simulink model "EV_Charger_SinglePhase_G2V"  (R2024b)
settings: Solver=ode23t  StartTime=0.0  StopTime=1  FixedStep=1e-6  RelTol=1e-3
undefined symbols (not defined in the file): Ion, Lithium
libraries: spsSeriesRLCBranchLib x8, spsMosfetLib x6, spsCurrentMeasurementLib x3, spsVoltageMeasurementLib x3, slpidlib x3, spsPLLLib x1, spsACVoltageSourceLib x1, spsPWMGeneratorDCDCLib x1, spsPWMGenerator2LevelLib x1, spsBatteryLib x1, sps_lib x1
settings Model: Creator=SUDHAK1  LastModifiedBy=SUDHAK1

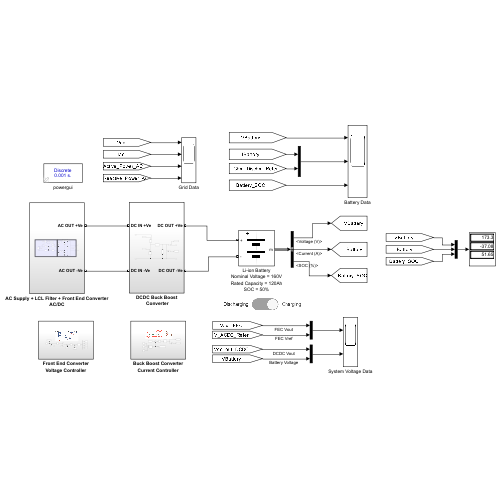
[thumbnail: Simulink's stored preview of the top-level diagram]
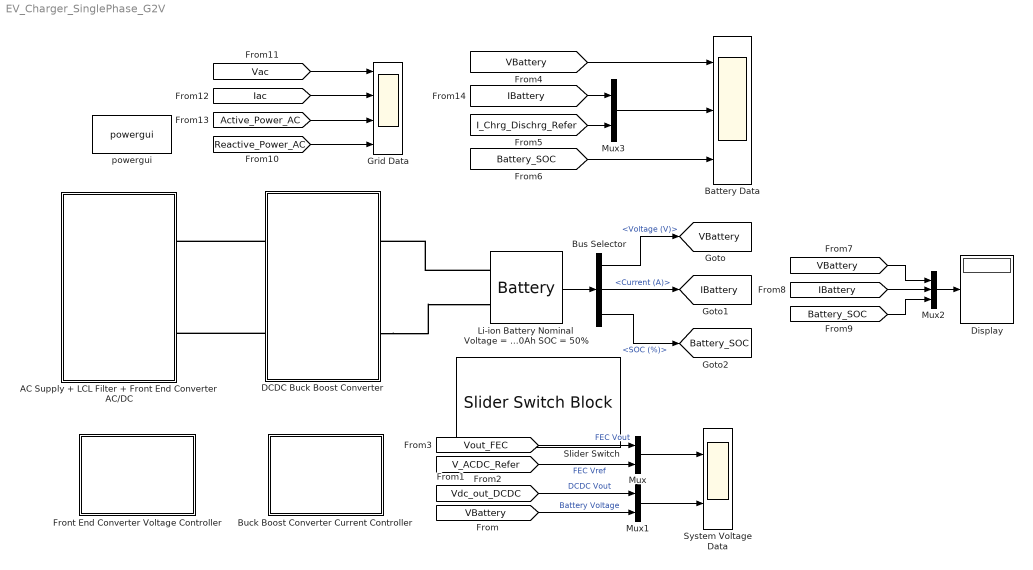
== system EV_Charger_SinglePhase_G2V ==
  AC Supply + LCL Filter + Front End Converter AC/DC : Subsystem
  Battery Data : Scope  NumInputPorts=3
  Buck Boost Converter Current Controller : Subsystem
  Bus Selector : BusSelector  OutputSignals=Voltage (V),Current (A),SOC (%)
  DCDC Buck Boost Converter : Subsystem
  Display : Display
  Front End Converter Voltage Controller : Subsystem
  Grid Data : Scope  NumInputPorts=4
  Li-ion Battery Nominal Voltage = 160V Rated Capacity = 120Ah SOC = 50% : spsBatteryLib/Battery  BatType=Lithium-Ion  NomV=160  NomQ=120  SOC=50  Batt_Tr=1  PresetModel=on  MaxQ=120  MinV=120  FullV=186.2379  Dis_rate=52.1739  R=0.013333  Normal_OP=108.5217  expZone="[172.8617      5.895652]"
  Mux : Mux  Inputs=2
  Mux1 : Mux  Inputs=2
  Mux2 : Mux  Inputs=3
  Mux3 : Mux  Inputs=2
  Slider Switch : SliderSwitchBlock  LabelPosition=Hide
      settings: Values={{'Discharging', 'Charging'}, [0 1]}
  System Voltage Data : Scope  NumInputPorts=2
  powergui : sps_lib/powergui  Priority=1  SimulationMode=Discrete  SampleTime=1e-3  frequency=60  Iterations=50  frequencyindice=50  Pbase=100e6  ErrMax=1e-4  UnitsV=kV  UnitsW=MW  buscounter=0  FunctionMessages=off  echomessages=off  EnableUseOfTLC=off  CurrentSourceSwitches=off  DisableSnubberDevices=off  DisableRonSwitches=off  DisableVfSwitches=off  DisplayEquations=off  AutomaticDiscreteSolvers=off  SolverType=Tustin/Backward Euler (TBE)  Interpol=off  ExternalGateDelay=off  methode=off  Ts=100  x0status=blocks  SPID=on  SwTol=0  HookPort=off  NonlinearTolerance=1e-4  nMaxIteration=100  ContinueOnMaxIteration=off  RestoreLinks=warning  ResistiveCurrentMeasurement=off  Frange=[0:2:500]  Ylog=off  Xlog=on  ShowGrid=off  save=off  variable=ZData  structure=0  ZoomFFT=off  StartTime=0.0  cycles=1  DisplayStyle=1  fundamental=60  FreqAxis=off  MaxFrequency=1000  frequencyindicesteady=1  RmsSteady=1  display=off
  tag scope: Battery_SOC=global, IBattery=global, VBattery=global
  wires:
  Li-ion Battery Nominal Voltage = 160V Rated Capacity = 120Ah SOC = 50%/1 -> Bus Selector/1
  Bus Selector/1 -> [VBattery]  "<Voltage (V)>"
  Bus Selector/2 -> [IBattery]  "<Current (A)>"
  Bus Selector/3 -> [Battery_SOC]  "<SOC (%)>"
  [VBattery] -> Mux2/1
  [Battery_SOC] -> Mux2/3
  [IBattery] -> Mux2/2
  Mux2/1 -> Display/1
  Mux/1 -> System Voltage Data/1
  [Vdc_out_DCDC] -> Mux1/1  "DCDC Vout"
  [VBattery] -> Mux1/2  "Battery Voltage"
  [V_ACDC_Refer] -> Mux/2  "FEC Vref"
  [Vout_FEC] -> Mux/1  "FEC Vout"
  [Reactive_Power_AC] -> Grid Data/4
  [VBattery] -> Battery Data/1
  [Vac] -> Grid Data/1
  [Battery_SOC] -> Battery Data/3
  [Active_Power_AC] -> Grid Data/3
  Mux1/1 -> System Voltage Data/2
  [Iac] -> Grid Data/2
  [IBattery] -> Mux3/1
  [I_Chrg_Dischrg_Refer] -> Mux3/2
  Mux3/1 -> Battery Data/2
  connections:
  Li-ion Battery Nominal Voltage = 160V Rated Capacity = 120Ah SOC = 50%/LConn1 -- DCDC Buck Boost Converter/RConn1
  DCDC Buck Boost Converter/RConn2 -- Li-ion Battery Nominal Voltage = 160V Rated Capacity = 120Ah SOC = 50%/LConn2
  DCDC Buck Boost Converter/LConn1 -- AC Supply + LCL Filter + Front End Converter AC/DC/RConn1
  DCDC Buck Boost Converter/LConn2 -- AC Supply + LCL Filter + Front End Converter AC/DC/RConn2

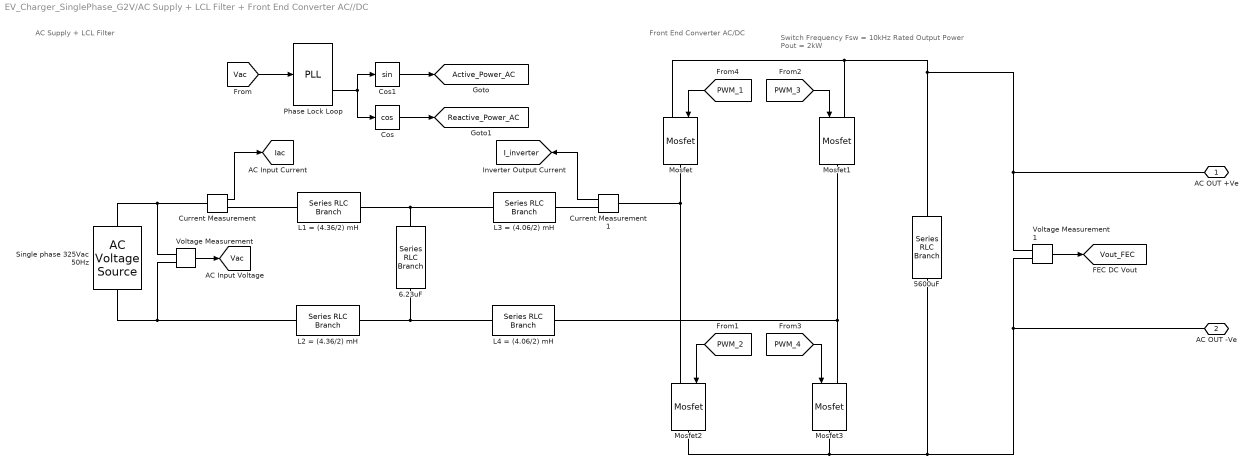
== system EV_Charger_SinglePhase_G2V/AC Supply + LCL Filter + Front End Converter AC//DC ==
  note: Front End Converter
      | AC/DC
  note: AC Supply + LCL Filter
  note: Switch Frequency Fsw = 10kHz
      | Rated Output Power Pout = 2kW
  5600uF : spsSeriesRLCBranchLib/Series RLC Branch  LConnTagsString=__new0  RConnTagsString=__new0  BranchType=RC  Resistance=0.0001  Inductance=1e-3  SetiL0=off  InitialCurrent=0  Capacitance=5600e-6  Setx0=on  InitialVoltage=400  Measurements=None
  6.23uF : spsSeriesRLCBranchLib/Series RLC Branch  LConnTagsString=__new0  RConnTagsString=__new0  BranchType=C  Resistance=1  Inductance=1e-3  SetiL0=off  InitialCurrent=0  Capacitance=6.23e-6  Setx0=off  InitialVoltage=0  Measurements=None
  Cos : Trigonometry  Operator=cos
  Cos1 : Trigonometry
  Current Measurement : spsCurrentMeasurementLib/Current Measurement  PhasorSimulation=off  OutputType=Complex  PSBequivalent=0
  Current Measurement1 : spsCurrentMeasurementLib/Current Measurement  PhasorSimulation=off  OutputType=Complex  PSBequivalent=0
  L1 = (4.36/2) mH : spsSeriesRLCBranchLib/Series RLC Branch  LConnTagsString=__new0  RConnTagsString=__new0  BranchType=L  Resistance=1  Inductance=4.36e-3/2  SetiL0=off  InitialCurrent=0  Capacitance=1e-6  Setx0=off  InitialVoltage=0  Measurements=None
  L2 = (4.36/2) mH : spsSeriesRLCBranchLib/Series RLC Branch  LConnTagsString=__new0  RConnTagsString=__new0  BranchType=L  Resistance=1  Inductance=4.36e-3/2  SetiL0=off  InitialCurrent=0  Capacitance=1e-6  Setx0=off  InitialVoltage=0  Measurements=None
  L3 = (4.06/2) mH : spsSeriesRLCBranchLib/Series RLC Branch  LConnTagsString=__new0  RConnTagsString=__new0  BranchType=L  Resistance=1  Inductance=4.06e-3/2  SetiL0=off  InitialCurrent=0  Capacitance=1e-6  Setx0=off  InitialVoltage=0  Measurements=None
  L4 = (4.06/2) mH : spsSeriesRLCBranchLib/Series RLC Branch  LConnTagsString=__new0  RConnTagsString=__new0  BranchType=L  Resistance=1  Inductance=4.06e-3/2  SetiL0=off  InitialCurrent=0  Capacitance=1e-6  Setx0=off  InitialVoltage=0  Measurements=None
  Mosfet{,1..3} (4 alike) : spsMosfetLib/Mosfet  Ron=0.1  Lon=0  Rd=0.01  Vfd=0  IC=0  Rs=1e5  Cs=inf  Measurements=off
  Phase Lock Loop : spsPLLLib/PLL  Fmin=45  Par_Init=[0, 50]  ParK=[180, 3200, 1]  TcD=1e-6  MaxRateChangeFreq=12  FilterCutOffFreq=25  Ts=0  AGC=on
      settings: LibrarySourceBlock=sps_lib/Control/PLL
  Single phase 325Vac 50Hz : spsACVoltageSourceLib/AC Voltage Source  Amplitude=325  Phase=0  Frequency=50  SampleTime=0  Measurements=None  BusType=swing  Pref=10e3  Qref=0  Qmin=-inf  Qmax=+inf
  Voltage Measurement : spsVoltageMeasurementLib/Voltage Measurement  PhasorSimulation=off  OutputType=Complex  PSBequivalent=0
  Voltage Measurement1 : spsVoltageMeasurementLib/Voltage Measurement  PhasorSimulation=off  OutputType=Complex  PSBequivalent=0
  AC OUT +Ve : PMIOPort  Side=Right
  AC OUT -Ve : PMIOPort  Port=2  Side=Right
  tag scope: Active_Power_AC=global, I_inverter=global, Iac=global, Reactive_Power_AC=global, Vac=global, Vout_FEC=global
  wires:
  Current Measurement1/1 -> [I_inverter]
  Current Measurement/1 -> [Iac]
  Voltage Measurement/1 -> [Vac]
  Voltage Measurement1/1 -> [Vout_FEC]
  [PWM_2] -> Mosfet2/1
  [PWM_1] -> Mosfet/1
  [PWM_3] -> Mosfet1/1
  [PWM_4] -> Mosfet3/1
  Phase Lock Loop/2 -> Cos1/1, Cos/1
  [Vac] -> Phase Lock Loop/1
  Cos/1 -> [Reactive_Power_AC]
  Cos1/1 -> [Active_Power_AC]
  connections:
  Current Measurement1/RConn1 -- L3 = (4.06/2) mH/RConn1
  Current Measurement/RConn1 -- L1 = (4.36/2) mH/LConn1
  L2 = (4.36/2) mH/RConn1 -- 6.23uF/RConn1 -- L4 = (4.06/2) mH/LConn1
  Single phase 325Vac 50Hz/LConn1 -- Voltage Measurement/LConn2 -- L2 = (4.36/2) mH/LConn1
  L1 = (4.36/2) mH/RConn1 -- 6.23uF/LConn1 -- L3 = (4.06/2) mH/LConn1
  Single phase 325Vac 50Hz/RConn1 -- Voltage Measurement/LConn1 -- Current Measurement/LConn1
  L4 = (4.06/2) mH/RConn1 -- Mosfet1/RConn1 -- Mosfet3/LConn1
  Current Measurement1/LConn1 -- Mosfet2/LConn1 -- Mosfet/RConn1
  5600uF/LConn1 -- Mosfet/LConn1 -- Mosfet1/LConn1 -- AC OUT +Ve/RConn1 -- Voltage Measurement1/LConn1
  5600uF/RConn1 -- Voltage Measurement1/LConn2 -- AC OUT -Ve/RConn1 -- Mosfet2/RConn1 -- Mosfet3/RConn1

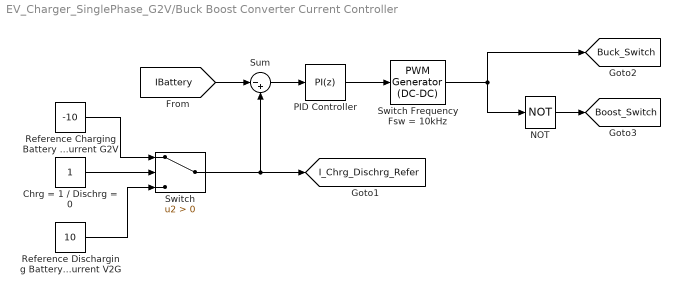
== system EV_Charger_SinglePhase_G2V/Buck Boost Converter Current Controller ==
  Chrg = 1 / Dischrg = 0 : Constant
  NOT : Logic  Operator=NOT  IconShape=distinctive  AllPortsSameDT=off  OutDataTypeStr=boolean
  PID Controller : slpidlib/PID Controller  Controller=PI  Form=Parallel  TimeDomain=Discrete-time  UseExternalTs=off  SampleTime=-1  IntegratorMethod=Forward Euler  FilterMethod=Forward Euler  ControllerParametersSource=internal  P=0.005  I=10  UseKiTs=off  D=0  UseExternalDerivativeSource=off  N=100  UseFilter=on  TunerSelectOption=Transfer Function Based (PID Tuner App)  InitialConditionSource=internal  InitialConditionForIntegrator=0  InitialConditionForFilter=0  DifferentiatorICPrevScaledInput=0  ExternalReset=none  TrackingMode=off  Kt=1  LimitOutput=on  SatLimitsSource=internal  UpperSaturationLimit=0.95  LowerSaturationLimit=0  LinearizeAsGain=on  AntiWindupMode=none  Kb=1  LimitIntegrator=off  UpperIntegratorSaturationLimit=inf  LowerIntegratorSaturationLimit=-inf  POutMin=[]  POutMax=[]  IOutMin=[]  IOutMax=[]  DOutMin=[]  DOutMax=[]  NOutMin=[]  NOutMax=[]  SumOutMin=[]  SumOutMax=[]  SaturationOutMin=[]  SaturationOutMax=[]  PParamMin=[]  PParamMax=[]  IParamMin=[]  IParamMax=[]  DParamMin=[]  DParamMax=[]  NParamMin=[]  NParamMax=[]  KbParamMin=[]  KbParamMax=[]  KtParamMin=[]  KtParamMax=[]  KbOutMin=[]  KbOutMax=[]  KtOutMin=[]  KtOutMax=[]  IntegratorOutMin=[]  IntegratorOutMax=[]  FilterOutMin=[]  FilterOutMax=[]  SumI1OutMin=[]  SumI1OutMax=[]  SumI2OutMin=[]  SumI2OutMax=[]  SumI3OutMin=[]  SumI3OutMax=[]  SumI4OutMin=[]  SumI4OutMax=[]  SumDOutMin=[]  SumDOutMax=[]  DifferentiatorOutMin=[]  DifferentiatorOutMax=[]  FilterDiffOutCoefMin=[]  FilterDiffOutCoefMax=[]  ReciprocalOutMin=[]  ReciprocalOutMax=[]  SumDenOutMin=[]  SumDenOutMax=[]  SumNumOutMin=[]  SumNumOutMax=[]  DivideOutMin=[]  DivideOutMax=[]  UdiffTsProdOutMin=[]  UdiffTsProdOutMax=[]  NTsProdOutMin=[]  NTsProdOutMax=[]  UintegralTsProdOutMin=[]  UintegralTsProdOutMax=[]  UngainTsProdOutMin=[]  UngainTsProdOutMax=[]  ClampingZeroOutDataTypeStr=Inherit: Inherit via back propagation  ClampingZeroOutMin=[]  ClampingZeroOutMax=[]  FilterDenConstantOutDataTypeStr=Inherit: Inherit via back propagation  FilterDenConstantOutMin=[]  FilterDenConstantOutMax=[]  PCopyOutDataTypeStr=Inherit: Inherit via back propagation  PCopyOutMin=[]  PCopyOutMax=[]  NCopyOutDataTypeStr=Inherit: Inherit via back propagation  NCopyOutMin=[]  NCopyOutMax=[]  IntegratorContinuousStateAttributes=''  IntegratorStateMustResolveToSignalObject=off  IntegratorRTWStateStorageClass=Auto  FilterContinuousStateAttributes=''  FilterStateMustResolveToSignalObject=off  FilterRTWStateStorageClass=Auto  ParallelPVariant=InternalParameters  IdealPVariant=Disabled  IVariant=InternalParameters  DVariant=Disabled  IntegratorVariant=Discrete  SatVariant=Enabled  AWVariant=Passthrough  PCopyVariant=Disabled  TRVariant=Disabled  FdbkBlocksVariant=Forward  IdealPFdbkVariant=Disabled  SatFdbkVariant=Disabled  DerivativeFilterVariant=Disabled  NVariant=Disabled  NCopyVariant=Disabled_SignalSpec  FilterICVariant=Disabled  IntegratorICVariant=InternalICs  ExternalResetVariant=Disabled  TRSumVariant=Passthrough  SumFdbkVariant=Disabled  SumVariant=Sum_PI  TsampFilterVariant=InternalTs  TsampNgainVariant=Passthrough  TsampIntegralVariant=Disabled_SignalSpec  ExternalSaturationOutDataTypeStr=Inherit: Same as second input  DerivativeSourceVariant=Disabled  PreIntVariant=InternalPreInt
  Reference Charging Battery Current G2V : Constant  Value=-10
  Reference Discharging Battery Current V2G : Constant  Value=10
  Sum : Sum  Inputs=|-+
  Switch : Switch  Criteria=u2 > Threshold  SaturateOnIntegerOverflow=off  InputSameDT=off
  Switch Frequency Fsw = 10kHz : spsPWMGeneratorDCDCLib/PWM Generator (DC-DC)  Fsw=10000  Ts=0
  tag scope: Boost_Switch=global, Buck_Switch=global, I_Chrg_Dischrg_Refer=global
  wires:
  PID Controller/1 -> Switch Frequency Fsw = 10kHz/1
  Switch Frequency Fsw = 10kHz/1 -> NOT/1, [Buck_Switch]
  NOT/1 -> [Boost_Switch]
  Sum/1 -> PID Controller/1
  [IBattery] -> Sum/1
  Reference Discharging Battery Current V2G/1 -> Switch/3
  Chrg = 1 / Dischrg = 0/1 -> Switch/2
  Reference Charging Battery Current G2V/1 -> Switch/1
  Switch/1 -> [I_Chrg_Dischrg_Refer], Sum/2

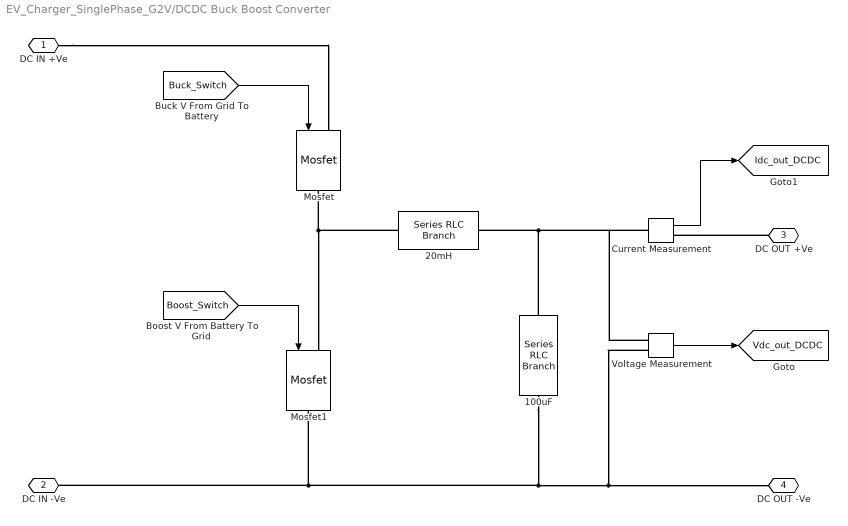
== system EV_Charger_SinglePhase_G2V/DCDC Buck Boost Converter ==
  100uF : spsSeriesRLCBranchLib/Series RLC Branch  LConnTagsString=__new0  RConnTagsString=__new0  BranchType=RC  Resistance=0.0001  Inductance=1e-3  SetiL0=off  InitialCurrent=0  Capacitance=100e-6  Setx0=off  InitialVoltage=0  Measurements=None
  20mH : spsSeriesRLCBranchLib/Series RLC Branch  LConnTagsString=__new0  RConnTagsString=__new0  BranchType=L  Resistance=1  Inductance=20e-3  SetiL0=off  InitialCurrent=0  Capacitance=1e-6  Setx0=off  InitialVoltage=0  Measurements=None
  Current Measurement : spsCurrentMeasurementLib/Current Measurement  PhasorSimulation=off  OutputType=Complex  PSBequivalent=0
  Mosfet : spsMosfetLib/Mosfet  Ron=0.1  Lon=0  Rd=0.01  Vfd=0  IC=0  Rs=1e5  Cs=inf  Measurements=off
  Mosfet1 : spsMosfetLib/Mosfet  Ron=0.1  Lon=0  Rd=0.01  Vfd=0  IC=0  Rs=1e5  Cs=inf  Measurements=off
  Voltage Measurement : spsVoltageMeasurementLib/Voltage Measurement  PhasorSimulation=off  OutputType=Complex  PSBequivalent=0
  DC IN +Ve : PMIOPort  Side=Left
  DC IN -Ve : PMIOPort  Port=2  Side=Left
  DC OUT +Ve : PMIOPort  Port=3  Side=Right
  DC OUT -Ve : PMIOPort  Port=4  Side=Right
  tag scope: Idc_out_DCDC=global, Vdc_out_DCDC=global
  wires:
  [Buck_Switch] -> Mosfet/1
  [Boost_Switch] -> Mosfet1/1
  Voltage Measurement/1 -> [Vdc_out_DCDC]
  Current Measurement/1 -> [Idc_out_DCDC]
  connections:
  100uF/LConn1 -- Current Measurement/LConn1 -- Voltage Measurement/LConn1 -- 20mH/RConn1
  100uF/RConn1 -- Voltage Measurement/LConn2 -- DC OUT -Ve/RConn1 -- DC IN -Ve/RConn1 -- Mosfet1/RConn1
  20mH/LConn1 -- Mosfet1/LConn1 -- Mosfet/RConn1
  DC IN +Ve/RConn1 -- Mosfet/LConn1
  DC OUT +Ve/RConn1 -- Current Measurement/RConn1

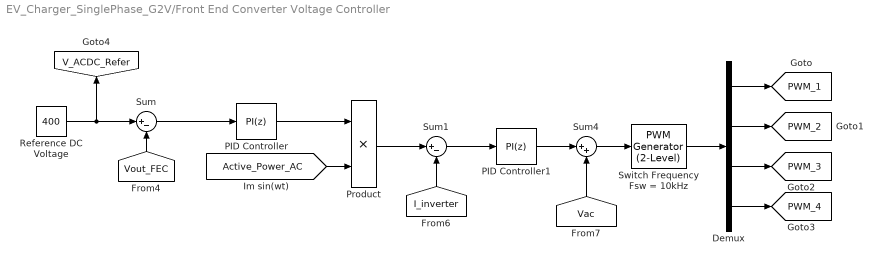
== system EV_Charger_SinglePhase_G2V/Front End Converter Voltage Controller ==
  Demux : Demux
  PID Controller : slpidlib/PID Controller  Controller=PI  Form=Parallel  TimeDomain=Discrete-time  UseExternalTs=off  SampleTime=-1  IntegratorMethod=Forward Euler  FilterMethod=Forward Euler  ControllerParametersSource=internal  P=1  I=10  UseKiTs=off  D=0  UseExternalDerivativeSource=off  N=100  UseFilter=on  TunerSelectOption=Transfer Function Based (PID Tuner App)  InitialConditionSource=internal  InitialConditionForIntegrator=0  InitialConditionForFilter=0  DifferentiatorICPrevScaledInput=0  ExternalReset=none  TrackingMode=off  Kt=1  LimitOutput=off  SatLimitsSource=internal  UpperSaturationLimit=inf  LowerSaturationLimit=-inf  LinearizeAsGain=on  AntiWindupMode=none  Kb=1  LimitIntegrator=off  UpperIntegratorSaturationLimit=inf  LowerIntegratorSaturationLimit=-inf  POutMin=[]  POutMax=[]  IOutMin=[]  IOutMax=[]  DOutMin=[]  DOutMax=[]  NOutMin=[]  NOutMax=[]  SumOutMin=[]  SumOutMax=[]  SaturationOutMin=[]  SaturationOutMax=[]  PParamMin=[]  PParamMax=[]  IParamMin=[]  IParamMax=[]  DParamMin=[]  DParamMax=[]  NParamMin=[]  NParamMax=[]  KbParamMin=[]  KbParamMax=[]  KtParamMin=[]  KtParamMax=[]  KbOutMin=[]  KbOutMax=[]  KtOutMin=[]  KtOutMax=[]  IntegratorOutMin=[]  IntegratorOutMax=[]  FilterOutMin=[]  FilterOutMax=[]  SumI1OutMin=[]  SumI1OutMax=[]  SumI2OutMin=[]  SumI2OutMax=[]  SumI3OutMin=[]  SumI3OutMax=[]  SumI4OutMin=[]  SumI4OutMax=[]  SumDOutMin=[]  SumDOutMax=[]  DifferentiatorOutMin=[]  DifferentiatorOutMax=[]  FilterDiffOutCoefMin=[]  FilterDiffOutCoefMax=[]  ReciprocalOutMin=[]  ReciprocalOutMax=[]  SumDenOutMin=[]  SumDenOutMax=[]  SumNumOutMin=[]  SumNumOutMax=[]  DivideOutMin=[]  DivideOutMax=[]  UdiffTsProdOutMin=[]  UdiffTsProdOutMax=[]  NTsProdOutMin=[]  NTsProdOutMax=[]  UintegralTsProdOutMin=[]  UintegralTsProdOutMax=[]  UngainTsProdOutMin=[]  UngainTsProdOutMax=[]  ClampingZeroOutDataTypeStr=Inherit: Inherit via back propagation  ClampingZeroOutMin=[]  ClampingZeroOutMax=[]  FilterDenConstantOutDataTypeStr=Inherit: Inherit via back propagation  FilterDenConstantOutMin=[]  FilterDenConstantOutMax=[]  PCopyOutDataTypeStr=Inherit: Inherit via back propagation  PCopyOutMin=[]  PCopyOutMax=[]  NCopyOutDataTypeStr=Inherit: Inherit via back propagation  NCopyOutMin=[]  NCopyOutMax=[]  IntegratorContinuousStateAttributes=''  IntegratorStateMustResolveToSignalObject=off  IntegratorRTWStateStorageClass=Auto  FilterContinuousStateAttributes=''  FilterStateMustResolveToSignalObject=off  FilterRTWStateStorageClass=Auto  ParallelPVariant=InternalParameters  IdealPVariant=Disabled  IVariant=InternalParameters  DVariant=Disabled  IntegratorVariant=Discrete  SatVariant=Disabled  AWVariant=Passthrough  PCopyVariant=Disabled  TRVariant=Disabled  FdbkBlocksVariant=Forward  IdealPFdbkVariant=Disabled  SatFdbkVariant=Disabled  DerivativeFilterVariant=Disabled  NVariant=Disabled  NCopyVariant=Disabled_SignalSpec  FilterICVariant=Disabled  IntegratorICVariant=InternalICs  ExternalResetVariant=Disabled  TRSumVariant=Passthrough  SumFdbkVariant=Disabled  SumVariant=Sum_PI  TsampFilterVariant=InternalTs  TsampNgainVariant=Passthrough  TsampIntegralVariant=Disabled_SignalSpec  ExternalSaturationOutDataTypeStr=Inherit: Same as second input  DerivativeSourceVariant=Disabled  PreIntVariant=InternalPreInt
  PID Controller1 : slpidlib/PID Controller  Controller=PI  Form=Parallel  TimeDomain=Discrete-time  UseExternalTs=off  SampleTime=-1  IntegratorMethod=Forward Euler  FilterMethod=Forward Euler  ControllerParametersSource=internal  P=10  I=100  UseKiTs=off  D=0  UseExternalDerivativeSource=off  N=100  UseFilter=on  TunerSelectOption=Transfer Function Based (PID Tuner App)  InitialConditionSource=internal  InitialConditionForIntegrator=0  InitialConditionForFilter=0  DifferentiatorICPrevScaledInput=0  ExternalReset=none  TrackingMode=off  Kt=1  LimitOutput=off  SatLimitsSource=internal  UpperSaturationLimit=inf  LowerSaturationLimit=-inf  LinearizeAsGain=on  AntiWindupMode=none  Kb=1  LimitIntegrator=off  UpperIntegratorSaturationLimit=inf  LowerIntegratorSaturationLimit=-inf  POutMin=[]  POutMax=[]  IOutMin=[]  IOutMax=[]  DOutMin=[]  DOutMax=[]  NOutMin=[]  NOutMax=[]  SumOutMin=[]  SumOutMax=[]  SaturationOutMin=[]  SaturationOutMax=[]  PParamMin=[]  PParamMax=[]  IParamMin=[]  IParamMax=[]  DParamMin=[]  DParamMax=[]  NParamMin=[]  NParamMax=[]  KbParamMin=[]  KbParamMax=[]  KtParamMin=[]  KtParamMax=[]  KbOutMin=[]  KbOutMax=[]  KtOutMin=[]  KtOutMax=[]  IntegratorOutMin=[]  IntegratorOutMax=[]  FilterOutMin=[]  FilterOutMax=[]  SumI1OutMin=[]  SumI1OutMax=[]  SumI2OutMin=[]  SumI2OutMax=[]  SumI3OutMin=[]  SumI3OutMax=[]  SumI4OutMin=[]  SumI4OutMax=[]  SumDOutMin=[]  SumDOutMax=[]  DifferentiatorOutMin=[]  DifferentiatorOutMax=[]  FilterDiffOutCoefMin=[]  FilterDiffOutCoefMax=[]  ReciprocalOutMin=[]  ReciprocalOutMax=[]  SumDenOutMin=[]  SumDenOutMax=[]  SumNumOutMin=[]  SumNumOutMax=[]  DivideOutMin=[]  DivideOutMax=[]  UdiffTsProdOutMin=[]  UdiffTsProdOutMax=[]  NTsProdOutMin=[]  NTsProdOutMax=[]  UintegralTsProdOutMin=[]  UintegralTsProdOutMax=[]  UngainTsProdOutMin=[]  UngainTsProdOutMax=[]  ClampingZeroOutDataTypeStr=Inherit: Inherit via back propagation  ClampingZeroOutMin=[]  ClampingZeroOutMax=[]  FilterDenConstantOutDataTypeStr=Inherit: Inherit via back propagation  FilterDenConstantOutMin=[]  FilterDenConstantOutMax=[]  PCopyOutDataTypeStr=Inherit: Inherit via back propagation  PCopyOutMin=[]  PCopyOutMax=[]  NCopyOutDataTypeStr=Inherit: Inherit via back propagation  NCopyOutMin=[]  NCopyOutMax=[]  IntegratorContinuousStateAttributes=''  IntegratorStateMustResolveToSignalObject=off  IntegratorRTWStateStorageClass=Auto  FilterContinuousStateAttributes=''  FilterStateMustResolveToSignalObject=off  FilterRTWStateStorageClass=Auto  ParallelPVariant=InternalParameters  IdealPVariant=Disabled  IVariant=InternalParameters  DVariant=Disabled  IntegratorVariant=Discrete  SatVariant=Disabled  AWVariant=Passthrough  PCopyVariant=Disabled  TRVariant=Disabled  FdbkBlocksVariant=Forward  IdealPFdbkVariant=Disabled  SatFdbkVariant=Disabled  DerivativeFilterVariant=Disabled  NVariant=Disabled  NCopyVariant=Disabled_SignalSpec  FilterICVariant=Disabled  IntegratorICVariant=InternalICs  ExternalResetVariant=Disabled  TRSumVariant=Passthrough  SumFdbkVariant=Disabled  SumVariant=Sum_PI  TsampFilterVariant=InternalTs  TsampNgainVariant=Passthrough  TsampIntegralVariant=Disabled_SignalSpec  ExternalSaturationOutDataTypeStr=Inherit: Same as second input  DerivativeSourceVariant=Disabled  PreIntVariant=InternalPreInt
  Product : Product
  Reference DC Voltage : Constant  Value=400
  Sum : Sum  Inputs=|+-
  Sum1 : Sum  Inputs=|+-
  Sum4 : Sum  Inputs=|++
  Switch Frequency Fsw = 10kHz : spsPWMGenerator2LevelLib/PWM Generator (2-Level)  ModulatorType=Single-phase full-bridge (4 pulses)  ModulatorMode=Unsynchronized  Fc=10000  Pc=90  nF=27  MinMax="[ 0  1 ]"  SamplingTechnique=Natural  ModulatingSignals=off  m=0.8  Freq=60  Phase=0  Ts=0  ShowCarrierOutport=off
  tag scope: PWM_1=global, PWM_2=global, PWM_3=global, PWM_4=global, V_ACDC_Refer=global
  wires:
  PID Controller1/1 -> Sum4/1
  Demux/4 -> [PWM_4]
  Sum1/1 -> PID Controller1/1
  Switch Frequency Fsw = 10kHz/1 -> Demux/1
  PID Controller/1 -> Product/1
  [Active_Power_AC] -> Product/2
  [I_inverter] -> Sum1/2
  Demux/3 -> [PWM_3]
  [Vac] -> Sum4/2
  Product/1 -> Sum1/1
  Demux/2 -> [PWM_2]
  Sum/1 -> PID Controller/1
  Demux/1 -> [PWM_1]
  Reference DC Voltage/1 -> Sum/1, [V_ACDC_Refer]
  Sum4/1 -> Switch Frequency Fsw = 10kHz/1
  [Vout_FEC] -> Sum/2
